simulink model "bf_flight_controller"  (R2025b)
settings: Solver=FixedStepDiscrete  StartTime=0.0  StopTime=t_sim  FixedStep=Ts  RelTol=1e-3
undefined symbols (not defined in the file or in its folder): Ts
settings Model: Creator=bmatt  LastModifiedBy=bmatt
settings ModelReferenceCC: ModelReferenceNumInstancesAllowed=Single
settings GRTTargetCC: SubcomponentCodeInterfacePackaging=Nonreusable function

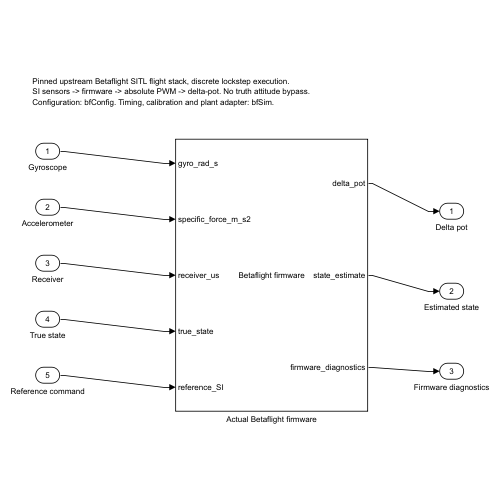
[thumbnail: Simulink's stored preview of the top-level diagram]
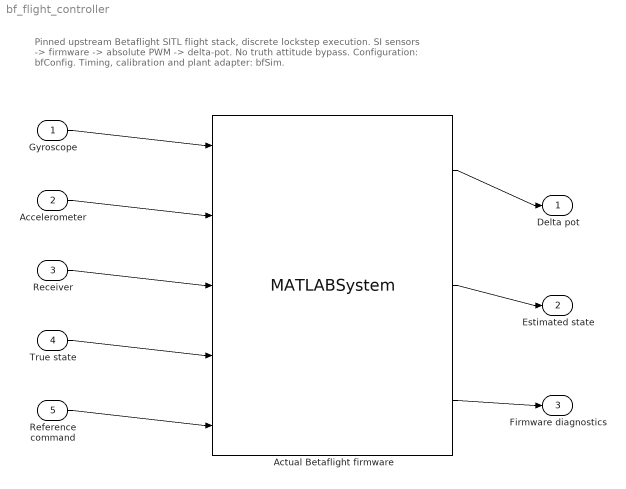
== system bf_flight_controller ==
  note: Pinned upstream Betaflight SITL flight stack, discrete lockstep execution.
      | SI sensors -> firmware -> absolute PWM -> delta-pot. No truth attitude bypass.
      | Configuration: bfConfig. Timing, calibration and plant adapter: bfSim.
  Gyroscope : Inport  PortDimensions=[3 1]  SampleTime=Ts
  Accelerometer : Inport  Port=2  PortDimensions=[3 1]  SampleTime=Ts
  Receiver : Inport  Port=3  PortDimensions=[16 1]  SampleTime=Ts
  True state : Inport  Port=4  PortDimensions=[12 1]  SampleTime=Ts
  Reference command : Inport  Port=5  PortDimensions=[12 1]  SampleTime=Ts
  Actual Betaflight firmware : MATLABSystem  System=bf.FlightController  Configuration=bfConfig  Options=bfSim  SampleTime=Ts  SimulateUsing=Interpreted execution
      mask Type: bf.FlightController
  Delta pot : Outport
  Estimated state : Outport  Port=2
  Firmware diagnostics : Outport  Port=3
  wires:
  Actual Betaflight firmware/1 -> Delta pot/1
  Actual Betaflight firmware/2 -> Estimated state/1
  Actual Betaflight firmware/3 -> Firmware diagnostics/1
  Gyroscope/1 -> Actual Betaflight firmware/1
  Accelerometer/1 -> Actual Betaflight firmware/2
  Receiver/1 -> Actual Betaflight firmware/3
  True state/1 -> Actual Betaflight firmware/4
  Reference command/1 -> Actual Betaflight firmware/5
